simulink model "complexCar"  (R2026a)
settings: Solver=VariableStepAuto
settings Model: Creator=sprinkle  LastModifiedBy=sprinkle

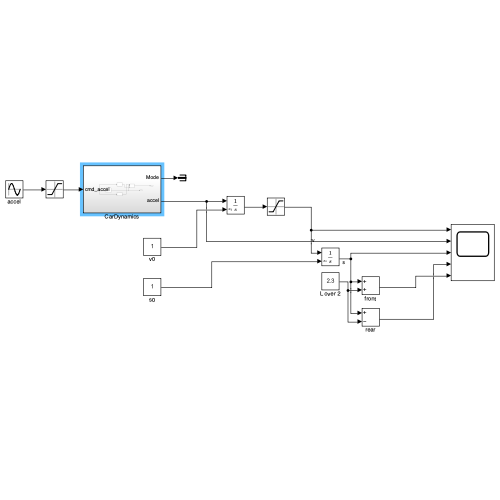
[thumbnail: Simulink's stored preview of the top-level diagram]
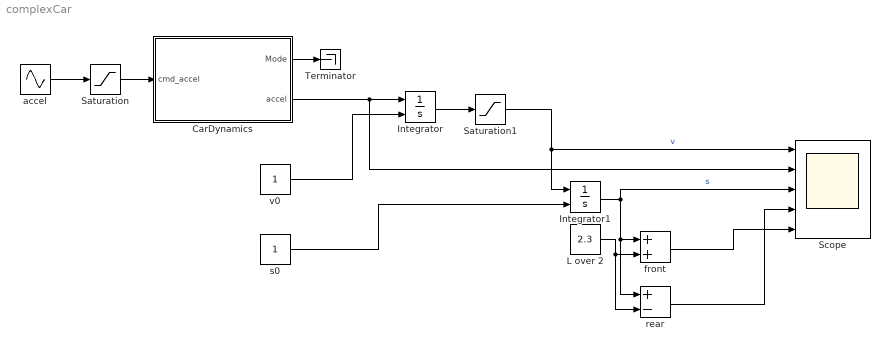
== system complexCar ==
  CarDynamics : Subsystem
  Integrator : Integrator  InitialConditionSource=external
  Integrator1 : Integrator  InitialConditionSource=external
  L over 2 : Constant  Value=2.3
  Saturation : Saturate  UpperLimit=1.5  LowerLimit=-3.5
  Saturation1 : Saturate  UpperLimit=30  LowerLimit=0
  Scope : Scope  NumInputPorts=5
      settings: ActiveDisplayYMinimum=-6.4319436824788268  ActiveDisplayYMaximum=22.887493142309445
  Terminator : Terminator
  accel : Sin  Amplitude=5  SampleTime=0
  front : Sum
  rear : Sum  Inputs=+-
  s0 : Constant
  v0 : Constant
  wires:
  Integrator/1 -> Saturation1/1
  v0/1 -> Integrator/2
  s0/1 -> Integrator1/2
  Integrator1/1 -> rear/1, front/1, Scope/3  "s"
  CarDynamics/2(accel) -> Scope/2, Integrator/1
  Saturation1/1 -> Integrator1/1, Scope/1  "v"
  L over 2/1 -> rear/2, front/2
  front/1 -> Scope/5
  rear/1 -> Scope/4
  accel/1 -> Saturation/1
  CarDynamics/1(Mode) -> Terminator/1
  Saturation/1 -> CarDynamics/1(cmd_accel)

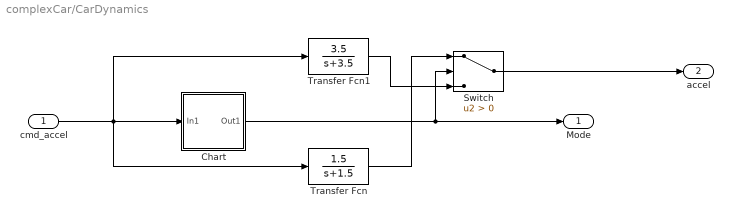
== system complexCar/CarDynamics ==
  cmd_accel : Inport
  Chart : Stateflow chart  TreatAsAtomicUnit=on
  Switch : Switch  Criteria=u2 > Threshold  SaturateOnIntegerOverflow=off  InputSameDT=off
  Transfer Fcn : TransferFcn  Numerator=[1.5]  Denominator=[1 1.5]
  Transfer Fcn1 : TransferFcn  Numerator=[3.5]  Denominator=[1 3.5]
  Mode : Outport
  accel : Outport  Port=2
  wires:
  cmd_accel/1 -> Chart/1(In1), Transfer Fcn/1, Transfer Fcn1/1
  Transfer Fcn1/1 -> Switch/3
  Switch/1 -> accel/1
  Transfer Fcn/1 -> Switch/1
  Chart/1(Out1) -> Mode/1, Switch/2

== stateflow chart complexCar/CarDynamics/Chart ==
  state Default
    entry: Out1=1;
  state Slowing
    entry: Out1=-1;
  (default) -> Default
  Slowing -> Default : [In1 > 0]
  Default -> Slowing : [In1 < 0.2]
  data: In1 input; Out1 output
